simulink model "My_gfm_battery_sil_1_Exciter_1"  (R2018b)
settings: Solver=ode23t  StartTime=0.0  StopTime=30  MaxStep=1e-4  RelTol=1e-3
PreLoadFcn:
  | modelDir = fileparts(get_param(bdroot,'FileName'));
  | 
  | load_system(fullfile(modelDir,'controls_element_lib.slx'));
  | load_system(fullfile(modelDir,'test_sequence_lib.slx'));
InitFcn:
  | close all;
  | clear all;
  | clc;
  | 
  | % frequency nominals
  | F_NOM = 60;
  | W_NOM = 2 * pi * F_NOM;
  | 
  | % base values relative to inverter
  | % --------------------------------
  | VLL_INV_NOM = 480;
  | P_INV_NOM = 1e6;
  | Q_INV_NOM = 0.5e6;
  | S_INV_NOM = sqrt(P_INV_NOM^2 + Q_INV_NOM^2);
  | 
  | I_INV_BASE = S_INV_NOM/(sqrt(3)*VLL_INV_NOM);
  | Z_INV_BASE = VLL_INV_NOM^2/S_INV_NOM;
  | L_INV_BASE = Z_INV_BASE / W_NOM;
  | C_INV_BASE = 1 / (Z_INV_BASE * W_NOM);
  | 
  | % nominal ratings for power system model
  | % --------------------------------------
  | INVERTER_COUNT = 100;
  | 
  | VLV_NOM = VLL_INV_NOM;
  | VMV_NOM = 35e3;
  | VHV_NOM = 230e3;
  | S_PLANT = INVERTER_COUNT * S_INV_NOM;
  | 
  | N_GSU = VHV_NOM/VMV_NOM;
  | N_MVT = VMV_NOM/VLV_NOM;
  | 
  | I_LV_BASE = S_PLANT/(sqrt(3)*VLV_NOM);
  | I_MV_BASE = S_PLANT/(sqrt(3)*VMV_NOM);
  | I_HV_BASE = S_PLANT/(sqrt(3)*VHV_NOM);
  | 
  | Z_LV_BASE = VLV_NOM^2/S_PLANT;
  | Z_MV_BASE = VMV_NOM^2/S_PLANT;
  | Z_HV_BASE = VHV_NOM^2/S_PLANT;
  | 
  | L_LV_BASE = Z_LV_BASE / W_NOM;
  | L_MV_BASE = Z_MV_BASE / W_NOM;
  | L_HV_BASE = Z_HV_BASE / W_NOM;
  | C_LV_BASE = 1 / (Z_LV_BASE * W_NOM);
  | C_MV_BASE = 1 / (Z_MV_BASE * W_NOM);
  | C_HV_BASE = 1 / (Z_HV_BASE * W_NOM);
undefined symbols (not defined in the file): j
libraries: simulink x38, test_sequence_lib x10, controls_element_lib x9
(part 6 of 6)

== system My_gfm_battery_sil_1_Exciter_1/My Inverter Controller /My_machineModel_A1/governer/synchronizer/assymmetric filter1 ==
  note: The saturation block is configured to cause a rapid rise, but much slow drop in output.
  in : Inport
  Gain1 : Gain  Gain=2
  Integrator : Integrator
  Saturation1 : Saturate  UpperLimit=VllRated  LowerLimit=-0.02 * VllRated
  Sum3 : Sum  Inputs=|+-
  out : Outport  VectorParamsAs1DForOutWhenUnconnected=on
  wires:
  Integrator/1 -> out/1, Sum3/2
  Sum3/1 -> Gain1/1
  in/1 -> Sum3/1
  Gain1/1 -> Saturation1/1
  Saturation1/1 -> Integrator/1

== system My_gfm_battery_sil_1_Exciter_1/My Inverter Controller /My_machineModel_A1/governer1/synchronizer/HPF ==
  in : Inport
  1/tau : Gain  Gain=2*pi*50
  Integrator : Integrator
  Sum : Sum  Inputs=|+-
  out : Outport  VectorParamsAs1DForOutWhenUnconnected=on
  wires:
  Sum/1 -> out/1, 1/tau/1
  in/1 -> Sum/1
  Integrator/1 -> Sum/2
  1/tau/1 -> Integrator/1

== system My_gfm_battery_sil_1_Exciter_1/My Inverter Controller /My_machineModel_A1/governer1/synchronizer/assymmetric filter1 ==
  note: The saturation block is configured to cause a rapid rise, but much slow drop in output.
  in : Inport
  Gain1 : Gain  Gain=2
  Integrator : Integrator
  Saturation1 : Saturate  UpperLimit=VllRated  LowerLimit=-0.02 * VllRated
  Sum3 : Sum  Inputs=|+-
  out : Outport  VectorParamsAs1DForOutWhenUnconnected=on
  wires:
  Integrator/1 -> out/1, Sum3/2
  Sum3/1 -> Gain1/1
  in/1 -> Sum3/1
  Gain1/1 -> Saturation1/1
  Saturation1/1 -> Integrator/1

== system My_gfm_battery_sil_1_Exciter_1/My Inverter Controller /My_machineModel_Other Exciter/governer/synchronizer/HPF  ==
  in : Inport
  Integrator : Integrator
  Sum : Sum  Inputs=|+-
  wSync : Gain  Gain=wSync
  out : Outport  VectorParamsAs1DForOutWhenUnconnected=on
  wires:
  Sum/1 -> out/1, wSync/1
  in/1 -> Sum/1
  Integrator/1 -> Sum/2
  wSync/1 -> Integrator/1

== system My_gfm_battery_sil_1_Exciter_1/My Inverter Controller /My_machineModel_Other Exciter/governer/synchronizer/assymmetric filter1 ==
  note: The saturation block is configured to cause a rapid rise, but much slow drop in output.
  in : Inport
  Gain1 : Gain  Gain=1/tauBkSt
  Integrator : Integrator
  Saturation1 : Saturate  UpperLimit=VllRated  LowerLimit=-0.02 * VllRated
  Sum3 : Sum  Inputs=|+-
  out : Outport  VectorParamsAs1DForOutWhenUnconnected=on
  wires:
  Integrator/1 -> out/1, Sum3/2
  Sum3/1 -> Gain1/1
  in/1 -> Sum3/1
  Gain1/1 -> Saturation1/1
  Saturation1/1 -> Integrator/1
